simulink model "YMBOX_Control_Core"  (R2024b)
settings: Solver=FixedStepDiscrete  StartTime=0.0  StopTime=3  RelTol=1e-3
PreLoadFcn:
  | run(fullfile(fileparts(get_param(bdroot,'FileName')), 'YMBOX_Deluxe_init.m'));
InitFcn:
  | YMBOX_InitializeModel('core',bdroot);
model workspace (MAT data in the model file):
  KuMDAS_ObserverBuildVariant : Simulink.Parameter (value not decoded)
undefined symbols (not defined in the file or in its folder): CeMDSM_DrvModeIfStart_enum, CeMDSM_DrvModeSpdSens_enum, CeMDSM_DrvModeSpdSmo_enum, CeMDSM_DrvModeTrq_enum, Cf_CONTROL_TASK_TIME_S, KbMDAS_SmoDeadTimeCompEnable_flg, KbMDSA_ActiveInverterCompEnable_flg, KbMDSA_UnifiedVoltageLimitEnable_flg, KbMDSP_DCBusVoltReportFilterEnable_flg, KbMDTM_DAxisPriorityInFW_flg, KbMDTM_FieldWeakeningEnable_flg, KbMDTM_FinalIqAntiWindupEnable_flg, KbMDTM_SensorlessFieldWeakeningEnable_flg, KbMDTM_TorquePriorityBelowBase_flg, KbMDTM_UnifiedConstraintEnable_flg, KfMDAS_ControlCountToElecRad_NULL, KfMDAS_IfAccel_rpms, KfMDAS_IfAlignTime_s, KfMDAS_IfBlendTime_s, KfMDAS_IfSwitchSpd_rpm, KfMDAS_NativeCountToMechRad_NULL, KfMDAS_ObserverExitRatio_NULL, KfMDAS_SlsCtrlPeriod_s, KfMDAS_SlsEAngleInit_rad, KfMDAS_SlsElecSpdMax_rads, KfMDAS_SlsElecSpdMin_rads, KfMDAS_SlsTwoPi_rad, KfMDAS_SmoAngleOffset_rad, KfMDAS_SmoCurrentZohCoefA_NULL, KfMDAS_SmoCurrentZohCoefB_AperV, KfMDAS_SmoDeadTimeCurrentBoundary_A, KfMDAS_SmoDeadTimeDuty_NULL, KfMDAS_SmoDeadTimePolarity_NULL, KfMDAS_SmoDeviceDrop_V, KfMDAS_SmoEmfLpfCoefA_NULL, KfMDAS_SmoEmfLpfCoefB_NULL, KfMDAS_SmoEmfLpfInvPole_s, KfMDAS_SmoErrBoundaryMax_A, KfMDAS_SmoErrBoundarySpan_A, KfMDAS_SmoGainSchedAlpha_NULL, KfMDAS_SmoGainSchedAngleComp_rad, KfMDAS_SmoGainSchedEmfLow_V, KfMDAS_SmoGainSchedInvSpan_PerV, KfMDAS_SmoLdMinusLq_H, KfMDAS_SmoPllKiTs_NULL, KfMDAS_SmoPllKp_NULL, KfMDAS_SmoPllMinEmf_V, KfMDAS_SmoPllSpeedLpfAlpha_NULL, KfMDAS_SmoSlideGainMin_V, KfMDAS_SmoSlideGainSpan_V, KfMDAS_SmoSwitchSpd_rpm, KfMDAS_SmoTotalDelay_s, KfMDCC_DqSoftwareOverCurrentThreshold_A, KfMDCC_PiKcTsId_NULL, KfMDCC_PiKcTsIq_NULL, KfMDCC_PiKiTsId_NULL, KfMDCC_PiKiTsIq_NULL, KfMDCC_PiKpValueId_NULL, KfMDCC_PiKpValueIq_NULL, KfMDCC_PwmFreq_Hz ... (+84)
libraries: YMBOX_SharedMath_Lib x11, spsabctoAlphaBetaZeroLib x1
(part 7 of 8)

== system YMBOX_Control_Core/MDSA/MDSA_Subsystem/PwmOutput/PwmEnable/SVM/SectorCalc/If Action Subsystem1 ==
  In2 : Inport
  In1 : Inport  Port=2
  Action Port : ActionPort  ActionPortLabel=else
  Constant : Constant  OutDataTypeStr=uint8
  Constant1 : Constant  Value=3  OutDataTypeStr=uint8
  Constant2 : Constant  Value=2  OutDataTypeStr=uint8
  Relational Operator : RelationalOperator  Operator=>  OutDataTypeStr=boolean  InputSameDT=off
  Relational Operator1 : RelationalOperator  Operator=<=  OutDataTypeStr=boolean  InputSameDT=off
  Switch : Switch  Criteria=u2 ~= 0  SaturateOnIntegerOverflow=off  InputSameDT=off
  Switch1 : Switch  Criteria=u2 ~= 0  SaturateOnIntegerOverflow=off  InputSameDT=off
  Unary Minus : UnaryMinus
  Out1 : Outport
  wires:
  Relational Operator1/1 -> Switch1/2
  Constant2/1 -> Switch1/3
  In2/1 -> Relational Operator/2, Unary Minus/1
  Switch/1 -> Out1/1
  Switch1/1 -> Switch/3
  Constant1/1 -> Switch1/1
  Unary Minus/1 -> Relational Operator1/2
  Relational Operator/1 -> Switch/2
  Constant/1 -> Switch/1
  In1/1 -> Relational Operator/1, Relational Operator1/1

== system YMBOX_Control_Core/MDSA/MDSA_Subsystem/PwmOutput/PwmEnable/SVM/T1T2CoefCalc/If Action Subsystem ==
  In1 : Inport
  In2 : Inport  Port=2
  Action Port : ActionPort  ActionPortLabel=if(u1 <= u2)
  Constant : Constant  OutDataTypeStr=single
  Out1 : Outport
  Out2 : Outport  Port=2
  Out3 : Outport  Port=3
  wires:
  Constant/1 -> Out3/1
  In2/1 -> Out2/1
  In1/1 -> Out1/1

== system YMBOX_Control_Core/MDSA/MDSA_Subsystem/PwmOutput/PwmEnable/SVM/T1T2CoefCalc/If Action Subsystem1 ==
  In1 : Inport
  In2 : Inport  Port=2
  Action Port : ActionPort  ActionPortLabel=else
  Add : Sum
  Constant : Constant  Value=KfMDSA_MaxDuty_NULL-KfMDSA_MinDuty_NULL  OutDataTypeStr=single
  Divide : Product  Inputs=**
  Divide1 : Product  Inputs=**
  Divide2 : Product  Inputs=*/
  Signal Conversion : SignalConversion  OverrideOpt=off
  Out1 : Outport
  Out2 : Outport  Port=2
  Out3 : Outport  Port=3
  wires:
  Signal Conversion/1 -> Out3/1
  Constant/1 -> Divide2/1
  Divide2/1 -> Divide/2, Divide1/2, Signal Conversion/1
  Add/1 -> Divide2/2
  Divide1/1 -> Out2/1
  Divide/1 -> Out1/1
  In2/1 -> Divide1/1, Add/2
  In1/1 -> Divide/1, Add/1

== system YMBOX_Control_Core/MDSA/MDSA_Subsystem/PwmOutput/PwmEnable/SVM/T1T2CoefCalc/Switch Case Action Subsystem ==
  VfMDSA_VoltAlpha_V : Inport
  VfMDSA_VoltBeta_V : Inport  Port=2
  VfMDSA_DCBusVolt_V : Inport  Port=3
  Action Port : ActionPort  ActionPortLabel=case [ 1 ]:
  Divide : Product  Inputs=*/
  Divide1 : Product  Inputs=*/
  Gain : Gain  Gain=1.5
  Gain1 : Gain  Gain=sqrt(3)/2
  Gain2 : Gain  Gain=sqrt(3)
  Subtract : Sum  Inputs=+-
  VfMDSA_tmpT1Coef_NULL : Outport
  VfMDSA_tmpT2Coef_NULL : Outport  Port=2
  wires:
  Gain2/1 -> Divide1/1
  Divide1/1 -> VfMDSA_tmpT2Coef_NULL/1
  Divide/1 -> VfMDSA_tmpT1Coef_NULL/1
  VfMDSA_DCBusVolt_V/1 -> Divide/2, Divide1/2
  Subtract/1 -> Divide/1
  Gain1/1 -> Subtract/2
  Gain/1 -> Subtract/1
  VfMDSA_VoltBeta_V/1 -> Gain1/1, Gain2/1
  VfMDSA_VoltAlpha_V/1 -> Gain/1

== system YMBOX_Control_Core/MDSA/MDSA_Subsystem/PwmOutput/PwmEnable/SVM/T1T2CoefCalc/Switch Case Action Subsystem1 ==
  VfMDSA_VoltAlpha_V : Inport
  VfMDSA_VoltBeta_V : Inport  Port=2
  VfMDSA_DCBusVolt_V : Inport  Port=3
  Action Port : ActionPort  ActionPortLabel=case [ 2 ]:
  Add : Sum
  Divide : Product  Inputs=*/
  Divide1 : Product  Inputs=*/
  Gain : Gain  Gain=sqrt(3)/2
  Gain1 : Gain  Gain=1.5
  Gain2 : Gain  Gain=1.5
  Gain3 : Gain  Gain=sqrt(3)/2
  Subtract : Sum  Inputs=+-
  VfMDSA_tmpT1Coef_NULL : Outport
  VfMDSA_tmpT2Coef_NULL : Outport  Port=2
  wires:
  Add/1 -> Divide1/1
  Gain3/1 -> Add/2
  Gain2/1 -> Add/1
  Gain1/1 -> Subtract/2
  Gain/1 -> Subtract/1
  Divide1/1 -> VfMDSA_tmpT2Coef_NULL/1
  Divide/1 -> VfMDSA_tmpT1Coef_NULL/1
  VfMDSA_DCBusVolt_V/1 -> Divide1/2, Divide/2
  Subtract/1 -> Divide/1
  VfMDSA_VoltBeta_V/1 -> Gain/1, Gain3/1
  VfMDSA_VoltAlpha_V/1 -> Gain1/1, Gain2/1

== system YMBOX_Control_Core/MDSA/MDSA_Subsystem/PwmOutput/PwmEnable/SVM/T1T2CoefCalc/Switch Case Action Subsystem2 ==
  VfMDSA_VoltAlpha_V : Inport
  VfMDSA_VoltBeta_V : Inport  Port=2
  VuMDSA_DCBusVolt_V : Inport  Port=3
  Action Port : ActionPort  ActionPortLabel=case [ 3 ]:
  Add : Sum
  Divide : Product  Inputs=*/
  Divide1 : Product  Inputs=*/
  Gain : Gain  Gain=sqrt(3)
  Gain1 : Gain  Gain=1.5
  Gain2 : Gain  Gain=sqrt(3)/2
  Unary Minus : UnaryMinus
  VfMDSA_tmpT1Coef_NULL : Outport
  VfMDSA_tmpT2Coef_NULL : Outport  Port=2
  wires:
  Unary Minus/1 -> Divide1/1
  Add/1 -> Unary Minus/1
  Gain/1 -> Divide/1
  Gain2/1 -> Add/2
  Gain1/1 -> Add/1
  Divide1/1 -> VfMDSA_tmpT2Coef_NULL/1
  Divide/1 -> VfMDSA_tmpT1Coef_NULL/1
  VuMDSA_DCBusVolt_V/1 -> Divide/2, Divide1/2
  VfMDSA_VoltBeta_V/1 -> Gain/1, Gain2/1
  VfMDSA_VoltAlpha_V/1 -> Gain1/1

== system YMBOX_Control_Core/MDSA/MDSA_Subsystem/PwmOutput/PwmEnable/SVM/T1T2CoefCalc/Switch Case Action Subsystem3 ==
  VfMDSA_VoltAlpha_V : Inport
  VfMDSA_VoltBeta_V : Inport  Port=2
  VfMDSA_DCBusVolt_V : Inport  Port=3
  Action Port : ActionPort  ActionPortLabel=case [ 4 ]:
  Divide : Product  Inputs=*/
  Divide1 : Product  Inputs=*/
  Gain : Gain  Gain=-sqrt(3)
  Gain1 : Gain  Gain=sqrt(3)/2
  Gain2 : Gain  Gain=1.5
  Subtract : Sum  Inputs=+-
  VfMDSA_tmpT1Coef_NULL : Outport
  VfMDSA_tmpT2Coef_NULL : Outport  Port=2
  wires:
  Subtract/1 -> Divide1/1
  Gain2/1 -> Subtract/2
  Gain1/1 -> Subtract/1
  Gain/1 -> Divide/1
  Divide1/1 -> VfMDSA_tmpT2Coef_NULL/1
  Divide/1 -> VfMDSA_tmpT1Coef_NULL/1
  VfMDSA_DCBusVolt_V/1 -> Divide/2, Divide1/2
  VfMDSA_VoltBeta_V/1 -> Gain/1, Gain1/1
  VfMDSA_VoltAlpha_V/1 -> Gain2/1

== system YMBOX_Control_Core/MDSA/MDSA_Subsystem/PwmOutput/PwmEnable/SVM/T1T2CoefCalc/Switch Case Action Subsystem4 ==
  VfMDSA_VoltAlpha_V : Inport
  VfMDSA_VoltBeta_V : Inport  Port=2
  VfMDSA_DCBusVolt_V : Inport  Port=3
  Action Port : ActionPort  ActionPortLabel=case [ 5 ]:
  Divide : Product  Inputs=*/
  Divide1 : Product  Inputs=*/
  Gain : Gain  Gain=1.5
  Gain1 : Gain  Gain=sqrt(3)/2
  Gain2 : Gain  Gain=sqrt(3)/2
  Gain3 : Gain  Gain=1.5
  Subtract : Sum
  Subtract1 : Sum  Inputs=+-
  Unary Minus : UnaryMinus
  VfMDSA_tmpT1Coef_NULL : Outport
  VfMDSA_tmpT2Coef_NULL : Outport  Port=2
  wires:
  Unary Minus/1 -> Divide/1
  Subtract1/1 -> Divide1/1
  Gain2/1 -> Subtract1/2
  Gain3/1 -> Subtract1/1
  Divide1/1 -> VfMDSA_tmpT2Coef_NULL/1
  Divide/1 -> VfMDSA_tmpT1Coef_NULL/1
  VfMDSA_DCBusVolt_V/1 -> Divide/2, Divide1/2
  Subtract/1 -> Unary Minus/1
  Gain1/1 -> Subtract/2
  Gain/1 -> Subtract/1
  VfMDSA_VoltBeta_V/1 -> Gain1/1, Gain2/1
  VfMDSA_VoltAlpha_V/1 -> Gain/1, Gain3/1

== system YMBOX_Control_Core/MDSA/MDSA_Subsystem/PwmOutput/PwmEnable/SVM/T1T2CoefCalc/Switch Case Action Subsystem5 ==
  VfMDSA_VoltAlpha_V : Inport
  VfMDSA_VoltBeta_V : Inport  Port=2
  VfMDSA_DCBusVolt_V : Inport  Port=3
  Action Port : ActionPort  ActionPortLabel=case [ 6 ]:
  Divide : Product  Inputs=*/
  Divide1 : Product  Inputs=*/
  Gain : Gain  Gain=1.5
  Gain1 : Gain  Gain=sqrt(3)/2
  Gain2 : Gain  Gain=-sqrt(3)
  Subtract : Sum
  VfMDSA_tmpT1Coef_NULL : Outport
  VfMDSA_tmpT2Coef_NULL : Outport  Port=2
  wires:
  Gain2/1 -> Divide1/1
  Divide1/1 -> VfMDSA_tmpT2Coef_NULL/1
  Divide/1 -> VfMDSA_tmpT1Coef_NULL/1
  VfMDSA_DCBusVolt_V/1 -> Divide/2, Divide1/2
  Subtract/1 -> Divide/1
  Gain1/1 -> Subtract/2
  Gain/1 -> Subtract/1
  VfMDSA_VoltBeta_V/1 -> Gain1/1, Gain2/1
  VfMDSA_VoltAlpha_V/1 -> Gain/1

== system YMBOX_Control_Core/MDSA/MDSA_Subsystem/PwmOutput/PwmEnable/SVM/TonUVWCal/Switch Case Action Subsystem ==
  VfMDSA_PwmDutyCyclePhaseA_NULL : Inport
  VfMDSA_PwmDutyCyclePhaseB_NULL : Inport  Port=2
  VfMDSA_PwmDutyCyclePhaseC_NULL : Inport  Port=3
  Action Port : ActionPort  ActionPortLabel=case [ 1 ]:
  VfMDSA_PwmDutyCyclePhaseU_NULL : Outport
  VfMDSA_PwmDutyCyclePhaseV_NULL : Outport  Port=2
  VfMDSA_PwmDutyCyclePhaseW_NULL : Outport  Port=3
  wires:
  VfMDSA_PwmDutyCyclePhaseC_NULL/1 -> VfMDSA_PwmDutyCyclePhaseW_NULL/1
  VfMDSA_PwmDutyCyclePhaseB_NULL/1 -> VfMDSA_PwmDutyCyclePhaseV_NULL/1
  VfMDSA_PwmDutyCyclePhaseA_NULL/1 -> VfMDSA_PwmDutyCyclePhaseU_NULL/1

== system YMBOX_Control_Core/MDSA/MDSA_Subsystem/PwmOutput/PwmEnable/SVM/TonUVWCal/Switch Case Action Subsystem1 ==
  VfMDSA_PwmDutyCyclePhaseA_NULL : Inport
  VfMDSA_PwmDutyCyclePhaseB_NULL : Inport  Port=2
  VfMDSA_PwmDutyCyclePhaseC_NULL1 : Inport  Port=3
  Action Port : ActionPort  ActionPortLabel=case [ 2 ]:
  VfMDSA_PwmDutyCyclePhaseU_NULL : Outport
  VfMDSA_PwmDutyCyclePhaseV_NULL : Outport  Port=2
  VfMDSA_PwmDutyCyclePhaseW_NULL : Outport  Port=3
  wires:
  VfMDSA_PwmDutyCyclePhaseA_NULL/1 -> VfMDSA_PwmDutyCyclePhaseV_NULL/1
  VfMDSA_PwmDutyCyclePhaseB_NULL/1 -> VfMDSA_PwmDutyCyclePhaseU_NULL/1
  VfMDSA_PwmDutyCyclePhaseC_NULL1/1 -> VfMDSA_PwmDutyCyclePhaseW_NULL/1

== system YMBOX_Control_Core/MDSA/MDSA_Subsystem/PwmOutput/PwmEnable/SVM/TonUVWCal/Switch Case Action Subsystem2 ==
  VfMDSA_PwmDutyCyclePhaseA_NULL : Inport
  VfMDSA_PwmDutyCyclePhaseB_NULL : Inport  Port=2
  VfMDSA_PwmDutyCyclePhaseC_NULL : Inport  Port=3
  Action Port : ActionPort  ActionPortLabel=case [ 3 ]:
  VfMDSA_PwmDutyCyclePhaseU_NULL : Outport
  VfMDSA_PwmDutyCyclePhaseV_NULL : Outport  Port=2
  VfMDSA_PwmDutyCyclePhaseW_NULL : Outport  Port=3
  wires:
  VfMDSA_PwmDutyCyclePhaseB_NULL/1 -> VfMDSA_PwmDutyCyclePhaseW_NULL/1
  VfMDSA_PwmDutyCyclePhaseA_NULL/1 -> VfMDSA_PwmDutyCyclePhaseV_NULL/1
  VfMDSA_PwmDutyCyclePhaseC_NULL/1 -> VfMDSA_PwmDutyCyclePhaseU_NULL/1

== system YMBOX_Control_Core/MDSA/MDSA_Subsystem/PwmOutput/PwmEnable/SVM/TonUVWCal/Switch Case Action Subsystem3 ==
  VfMDSA_PwmDutyCyclePhaseA_NULL : Inport
  VfMDSA_PwmDutyCyclePhaseB_NULL : Inport  Port=2
  VfMDSA_PwmDutyCyclePhaseC_NULL : Inport  Port=3
  Action Port : ActionPort  ActionPortLabel=case [ 4 ]:
  VfMDSA_PwmDutyCyclePhaseU_NULL : Outport
  VfMDSA_PwmDutyCyclePhaseV_NULL : Outport  Port=2
  VfMDSA_PwmDutyCyclePhaseW_NULL : Outport  Port=3
  wires:
  VfMDSA_PwmDutyCyclePhaseA_NULL/1 -> VfMDSA_PwmDutyCyclePhaseW_NULL/1
  VfMDSA_PwmDutyCyclePhaseB_NULL/1 -> VfMDSA_PwmDutyCyclePhaseV_NULL/1
  VfMDSA_PwmDutyCyclePhaseC_NULL/1 -> VfMDSA_PwmDutyCyclePhaseU_NULL/1

== system YMBOX_Control_Core/MDSA/MDSA_Subsystem/PwmOutput/PwmEnable/SVM/TonUVWCal/Switch Case Action Subsystem4 ==
  VfMDSA_PwmDutyCyclePhaseA_NULL : Inport
  VfMDSA_PwmDutyCyclePhaseB_NULL : Inport  Port=2
  VfMDSA_PwmDutyCyclePhaseC_NULL : Inport  Port=3
  Action Port : ActionPort  ActionPortLabel=case [ 5 ]:
  VfMDSA_PwmDutyCyclePhaseU_NULL : Outport
  VfMDSA_PwmDutyCyclePhaseV_NULL : Outport  Port=2
  VfMDSA_PwmDutyCyclePhaseW_NULL : Outport  Port=3
  wires:
  VfMDSA_PwmDutyCyclePhaseA_NULL/1 -> VfMDSA_PwmDutyCyclePhaseW_NULL/1
  VfMDSA_PwmDutyCyclePhaseC_NULL/1 -> VfMDSA_PwmDutyCyclePhaseV_NULL/1
  VfMDSA_PwmDutyCyclePhaseB_NULL/1 -> VfMDSA_PwmDutyCyclePhaseU_NULL/1

== system YMBOX_Control_Core/MDSA/MDSA_Subsystem/PwmOutput/PwmEnable/SVM/TonUVWCal/Switch Case Action Subsystem5 ==
  VfMDSA_PwmDutyCyclePhaseA_NULL : Inport
  VfMDSA_PwmDutyCyclePhaseB_NULL : Inport  Port=2
  VfMDSA_PwmDutyCyclePhaseC_NULL : Inport  Port=3
  Action Port : ActionPort  ActionPortLabel=case [ 6 ]:
  VfMDSA_PwmDutyCyclePhaseU_NULL : Outport
  VfMDSA_PwmDutyCyclePhaseV_NULL : Outport  Port=2
  VfMDSA_PwmDutyCyclePhaseW_NULL : Outport  Port=3
  wires:
  VfMDSA_PwmDutyCyclePhaseB_NULL/1 -> VfMDSA_PwmDutyCyclePhaseW_NULL/1
  VfMDSA_PwmDutyCyclePhaseC_NULL/1 -> VfMDSA_PwmDutyCyclePhaseV_NULL/1
  VfMDSA_PwmDutyCyclePhaseA_NULL/1 -> VfMDSA_PwmDutyCyclePhaseU_NULL/1

== stateflow chart YMBOX_Control_Core/Control_Task_Dispatcher/Scheduler ==
  settings: sampleTime=50e-6
  (default) -> (junction 78) : {
      |   trig_MDSP_ControlTask;
      |   trig_MDFM_ControlTask;
      |   trig_MDSM_ControlTask;
      |   trig_MDAS_ControlTask;
      |   VuMDTM_DividerCount_NULL = VuMDTM_DividerCount_NULL + 1;
      | }
  (junction 78) -> (junction 80) [order 2]
  (junction 78) -> (junction 79) [order 1] : [VuMDTM_DividerCount_NULL >= KuMDTM_TaskDivider_NULL || MDTM_ResetDispatch]
      | {
      |  VuMDTM_DividerCount_NULL = 0;
      |  trig_MDTM_ControlTask;
      | }
  (junction 80) -> (junction 68) : {
      |   trig_MDCC_ControlTask;
      |   trig_MDSA_ControlTask;
      | }
  (junction 79) -> (junction 68) : {
      |   trig_MDCC_ControlTask;
      |   trig_MDSA_ControlTask;
      | }
  data: KuMDTM_TaskDivider_NULL parameter uint16; VuMDTM_DividerCount_NULL local uint16; MDTM_ResetDispatch data_store_memory
  events: trig_MDFM_ControlTask output FUNCTION_CALL_EVENT; trig_MDSM_ControlTask output FUNCTION_CALL_EVENT; trig_MDAS_ControlTask output FUNCTION_CALL_EVENT; trig_MDTM_ControlTask output FUNCTION_CALL_EVENT; trig_MDCC_ControlTask output FUNCTION_CALL_EVENT; trig_MDSA_ControlTask output FUNCTION_CALL_EVENT; trig_MDSP_ControlTask output FUNCTION_CALL_EVENT

== stateflow chart YMBOX_Control_Core/MDSM/MDSM_ModeManager/MDSM_Supervisor_Variant/MDSM_Supervisor_SMO/MDSM_GenericSupervisor ==
  settings: description=INDUSTRIAL_SENSORLESS_V6. Generic runtime supervisor. The compile-time Variant route table supplies observer identity, qualification, threshold, acquisition dwell and optional fallback. Stateflow only supervises I/F, STAGE1 and optional STAGE2.
  state OFF
    entry:
    VeMDSM_DrvModeCmd_enum=0; VuMDSM_StateDwell_cnt=0;
    VbMDTM_PiReset_flg=1; VbMDCC_PiReset_flg=1; VuMDFM_FFEnable_enum=0;
    during:
    VeMDSM_DrvModeCmd_enum=0; VuMDSM_StateDwell_cnt=0;
    VbMDTM_PiReset_flg=0; VbMDCC_PiReset_flg=0; VuMDFM_FFEnable_enum=0;
  state DIRECT
    entry:
    VeMDSM_ActiveDirectMode_enum=VeMDSM_DrvModeReq_enum;
    VeMDSM_DrvModeCmd_enum=VeMDSM_ActiveDirectMode_enum; VuMDSM_StateDwell_cnt=0;
    VbMDTM_PiReset_flg=1; VbMDCC_PiReset_flg=1; VuMDFM_FFEnable_enum=(VeMDSM_ActiveDirectMode_enum>=3)*KuMDCC_VoltageFFMode_enum;
    during:
    VbMDTM_PiReset_flg=(VeMDSM_DrvModeReq_enum!=VeMDSM_ActiveDirectMode_enum);
    VbMDCC_PiReset_flg=VbMDTM_PiReset_flg;
    VeMDSM_ActiveDirectMode_enum=VeMDSM_DrvModeReq_enum;
    VeMDSM_DrvModeCmd_enum=VeMDSM_ActiveDirectMode_enum; VuMDSM_StateDwell_cnt=0; VuMDFM_FFEnable_enum=(VeMDSM_ActiveDirectMode_enum>=3)*KuMDCC_VoltageFFMode_enum;
  state SENSORLESS
    state IF_RAMP
      entry:
      VeMDSM_DrvModeCmd_enum=16; VuMDSM_StateDwell_cnt=0; VuMDFM_FFEnable_enum=KuMDCC_VoltageFFMode_enum;
      during:
      VeMDSM_DrvModeCmd_enum=16;
      VuMDSM_StateDwell_cnt=VuMDSM_StateDwell_cnt+1;
      VbMDTM_PiReset_flg=0; VbMDCC_PiReset_flg=0; VuMDFM_FFEnable_enum=KuMDCC_VoltageFFMode_enum;
    state SMO_ACTIVE
      entry:
      VeMDSM_DrvModeCmd_enum=VeMDSM_Stage1Mode_enum; VuMDSM_StateDwell_cnt=0;
      VuMDSM_AcquireElapsed_cnt=VuMDSM_AcquireElapsed_cnt+(VuMDSM_AcquireElapsed_cnt<VuMDSM_Stage1Acquire_cnt);
      VuMDFM_FFEnable_enum=KuMDCC_VoltageFFMode_enum;
      during:
      VeMDSM_DrvModeCmd_enum=VeMDSM_Stage1Mode_enum;
      VuMDSM_AcquireElapsed_cnt=VuMDSM_AcquireElapsed_cnt+(VuMDSM_AcquireElapsed_cnt<VuMDSM_Stage1Acquire_cnt);
      VbMDTM_PiReset_flg=0; VbMDCC_PiReset_flg=0; VuMDFM_FFEnable_enum=KuMDCC_VoltageFFMode_enum;
    state SMO_LOSS_CONFIRM
      entry:
      VeMDSM_DrvModeCmd_enum=VeMDSM_Stage1Mode_enum; VuMDSM_StateDwell_cnt=1;
      VuMDSM_AcquireElapsed_cnt=VuMDSM_AcquireElapsed_cnt+(VuMDSM_AcquireElapsed_cnt<VuMDSM_Stage1Acquire_cnt);
      VbMDTM_PiReset_flg=0; VbMDCC_PiReset_flg=0; VuMDFM_FFEnable_enum=KuMDCC_VoltageFFMode_enum;
      during:
      VeMDSM_DrvModeCmd_enum=VeMDSM_Stage1Mode_enum;
      VuMDSM_StateDwell_cnt=VuMDSM_StateDwell_cnt+(VuMDSM_StateDwell_cnt<KuMDSM_ObserverLossConfirmCnt);
      VuMDSM_AcquireElapsed_cnt=VuMDSM_AcquireElapsed_cnt+(VuMDSM_AcquireElapsed_cnt<VuMDSM_Stage1Acquire_cnt);
      VbMDTM_PiReset_flg=0; VbMDCC_PiReset_flg=0; VuMDFM_FFEnable_enum=KuMDCC_VoltageFFMode_enum;
    state SENSORLESS_FAULT
      entry:
      VeMDSM_DrvModeCmd_enum=0; VuMDSM_StateDwell_cnt=0;
      VbMDTM_PiReset_flg=1; VbMDCC_PiReset_flg=1; VuMDFM_FFEnable_enum=0;
      during:
      VeMDSM_DrvModeCmd_enum=0; VuMDSM_StateDwell_cnt=0;
      VbMDTM_PiReset_flg=0; VbMDCC_PiReset_flg=0; VuMDFM_FFEnable_enum=0;
    state IF_LOW_SPEED
      entry:
      VeMDSM_DrvModeCmd_enum=16; VuMDSM_StateDwell_cnt=0;
      VbMDTM_PiReset_flg=1; VbMDCC_PiReset_flg=1; VuMDFM_FFEnable_enum=KuMDCC_VoltageFFMode_enum;
      during:
      VeMDSM_DrvModeCmd_enum=16; VuMDSM_StateDwell_cnt=0;
      VbMDTM_PiReset_flg=0; VbMDCC_PiReset_flg=0; VuMDFM_FFEnable_enum=KuMDCC_VoltageFFMode_enum;
    (default) -> IF_RAMP : /VbMDTM_PiReset_flg=1; VbMDCC_PiReset_flg=1;
    IF_RAMP -> SENSORLESS_FAULT [order 3] : [abs(VfMDSM_TrgtSpd_rpm)>=VfMDSM_Stage1SwitchSpd_rpm && VbMDSM_Stage1Ready_flg==0 && VuMDSM_StateDwell_cnt>=KuMDSM_IFStartupTimeoutCnt]
    IF_RAMP -> SMO_ACTIVE [order 2] : [abs(VfMDSM_TrgtSpd_rpm)>=VfMDSM_Stage1SwitchSpd_rpm && VbMDSM_Stage1Ready_flg!=0]/VuMDSM_AcquireElapsed_cnt=0; VbMDTM_PiReset_flg=1; VbMDCC_PiReset_flg=0;
    SMO_LOSS_CONFIRM -> IF_RAMP [order 3] : [VuMDSM_StateDwell_cnt>=KuMDSM_ObserverLossConfirmCnt && VuMDSM_AcquireElapsed_cnt<VuMDSM_Stage1Acquire_cnt]/VbMDTM_PiReset_flg=0; VbMDCC_PiReset_flg=0;
    IF_RAMP -> IF_LOW_SPEED [order 1] : [abs(VfMDSM_TrgtSpd_rpm)<VfMDSM_Stage1SwitchSpd_rpm]
    IF_LOW_SPEED -> IF_RAMP : [abs(VfMDSM_TrgtSpd_rpm)>=VfMDSM_Stage1SwitchSpd_rpm]/VbMDTM_PiReset_flg=0; VbMDCC_PiReset_flg=0;
    SMO_ACTIVE -> SMO_LOSS_CONFIRM : [VbMDSM_Stage1Ready_flg==0]
    SMO_LOSS_CONFIRM -> SMO_ACTIVE [order 1] : [VbMDSM_Stage1Ready_flg!=0]/VbMDTM_PiReset_flg=0; VbMDCC_PiReset_flg=0;
    SMO_LOSS_CONFIRM -> SENSORLESS_FAULT [order 4] : [VuMDSM_StateDwell_cnt>=KuMDSM_ObserverLossConfirmCnt && VuMDSM_AcquireElapsed_cnt>=VuMDSM_Stage1Acquire_cnt]
    SMO_LOSS_CONFIRM -> IF_LOW_SPEED [order 2] : [VuMDSM_StateDwell_cnt>=KuMDSM_ObserverLossConfirmCnt && abs(VfMDSM_TrgtSpd_rpm)<KfMDAS_ObserverExitRatio_NULL*VfMDSM_Stage1SwitchSpd_rpm]
  (default) -> OFF
  DIRECT -> OFF [order 1] : [VbMDSM_MCUEnb_flg==0 || VeMDSM_DrvModeReq_enum==0 || VeMDSM_DrvModeReq_enum>6]
  OFF -> DIRECT [order 1] : [VbMDSM_MCUEnb_flg!=0 && VeMDSM_DrvModeReq_enum>=1 && VeMDSM_DrvModeReq_enum<=5]
  SENSORLESS -> OFF [order 1] : [VbMDSM_MCUEnb_flg==0 || VeMDSM_DrvModeReq_enum==0 || VeMDSM_DrvModeReq_enum>6]
  OFF -> SENSORLESS [order 2] : [VbMDSM_MCUEnb_flg!=0 && VeMDSM_DrvModeReq_enum==6]
  SENSORLESS -> DIRECT [order 2] : [VbMDSM_MCUEnb_flg!=0 && VeMDSM_DrvModeReq_enum>=1 && VeMDSM_DrvModeReq_enum<=5]
  DIRECT -> SENSORLESS [order 2] : [VbMDSM_MCUEnb_flg!=0 && VeMDSM_DrvModeReq_enum==6]
  data: VeMDSM_DrvModeReq_enum input; VbMDSM_MCUEnb_flg input; VbMDSM_RouteSupported_flg input; VeMDSM_Stage1Mode_enum input; VbMDSM_Stage1Ready_flg input; VfMDSM_Stage1SwitchSpd_rpm input; VuMDSM_Stage1Acquire_cnt input; VbMDSM_Stage2Enable_flg input; VeMDSM_Stage2Mode_enum input; VbMDSM_Stage2Ready_flg input; VfMDSM_Stage2SwitchSpd_rpm input; VbMDSM_Stage2Fallback_flg input; VfMDSM_TrgtSpd_rpm input; VeMDSM_DrvModeCmd_enum output uint16; VbMDTM_PiReset_flg output boolean; VbMDCC_PiReset_flg output boolean; VuMDFM_FFEnable_enum output uint8; KuMDSM_ObserverLossConfirmCnt parameter uint32; KuMDSM_IFStartupTimeoutCnt parameter uint32; KfMDAS_ObserverExitRatio_NULL parameter single; VeMDSM_ActiveDirectMode_enum local uint16; VuMDSM_StateDwell_cnt local uint32; KuMDCC_VoltageFFMode_enum parameter uint8; VuMDSM_AcquireElapsed_cnt local uint32

== stateflow chart YMBOX_Control_Core/MDAS/IF_Startup_Internal/IF_Startup_SMO/SMO_ProductMode_Core ==
  state RunSMOProductMode
    en:
    [VfMDAS_IfMechSpd_rads, VfMDAS_IfMechSpdAbs_rads, ...
    VfMDAS_IfElecAngle_rad, VfMDAS_SmoMechSpd_rads, ...
    VfMDAS_SmoMechSpdAbs_rads, VbMDAS_SmoReady_flg, ...
    VfMDAS_SmoAlignedElecAngle_rad, VfMDAS_HandoverBlend_NULL, ...
    VfMDAS_HandoverElecAngleDelta_rad] = YMBOX_SmoProductModeCore( ...
    VeMDAS_DrvModeCmd_enum, VeMDAS_DrvModeReq_enum, ...
    VfMDAS_TargetSpd_rpm, VfMDAS_SmoElecSpd_rads, ...
    VfMDAS_SmoElecAngle_rad, VfMDAS_SmoEmfMag_V, ...
    VfMDAS_SmoPllPhaseErr_NULL, KfMDAS_SlsCtrlPeriod_s, ...
    KuMDMP_Pole_Pair_Number_NULL, KfMDAS_IfAccel_rpms, ...
    KfMDAS_IfAccelBlendTime_s, KfMDAS_IfAlignTime_s, ...
    KfMDAS_IfBlendTime_s, KfMDAS_SmoSwitchSpd_rpm, ...
    KfMDAS_SmoReadySpdErr_rads, KfMDAS_SmoReadyPllErr_NULL, ...
    KuMDAS_SmoReadyConfirmCnt, KfMDAS_SmoPllMinEmf_V, ...
    KfMDAS_DirectHandoverTime_s, KfMDAS_ObserverExitRatio_NULL);
    du:
    [VfMDAS_IfMechSpd_rads, VfMDAS_IfMechSpdAbs_rads, ...
    VfMDAS_IfElecAngle_rad, VfMDAS_SmoMechSpd_rads, ...
    VfMDAS_SmoMechSpdAbs_rads, VbMDAS_SmoReady_flg, ...
    VfMDAS_SmoAlignedElecAngle_rad, VfMDAS_HandoverBlend_NULL, ...
    VfMDAS_HandoverElecAngleDelta_rad] = YMBOX_SmoProductModeCore( ...
    VeMDAS_DrvModeCmd_enum, VeMDAS_DrvModeReq_enum, ...
    VfMDAS_TargetSpd_rpm, VfMDAS_SmoElecSpd_rads, ...
    VfMDAS_SmoElecAngle_rad, VfMDAS_SmoEmfMag_V, ...
    VfMDAS_SmoPllPhaseErr_NULL, KfMDAS_SlsCtrlPeriod_s, ...
    KuMDMP_Pole_Pair_Number_NULL, KfMDAS_IfAccel_rpms, ...
    KfMDAS_IfAccelBlendTime_s, KfMDAS_IfAlignTime_s, ...
    KfMDAS_IfBlendTime_s, KfMDAS_SmoSwitchSpd_rpm, ...
    KfMDAS_SmoReadySpdErr_rads, KfMDAS_SmoReadyPllErr_NULL, ...
    KuMDAS_SmoReadyConfirmCnt, KfMDAS_SmoPllMinEmf_V, ...
    KfMDAS_DirectHandoverTime_s, KfMDAS_ObserverExitRatio_NULL);
  (default) -> RunSMOProductMode
  data: VeMDAS_DrvModeCmd_enum input uint16; VeMDAS_DrvModeReq_enum input uint16; VfMDAS_TargetSpd_rpm input single; VfMDAS_SmoElecSpd_rads input single; VfMDAS_SmoElecAngle_rad input single; VfMDAS_SmoEmfMag_V input single; VfMDAS_SmoPllPhaseErr_NULL input single; VfMDAS_IfMechSpd_rads output single; VfMDAS_IfMechSpdAbs_rads output single; VfMDAS_IfElecAngle_rad output single; VfMDAS_SmoMechSpd_rads output single; VfMDAS_SmoMechSpdAbs_rads output single; VbMDAS_SmoReady_flg output boolean; VfMDAS_SmoAlignedElecAngle_rad output single; VfMDAS_HandoverBlend_NULL output single; VfMDAS_HandoverElecAngleDelta_rad output single; KfMDAS_SlsCtrlPeriod_s parameter single; KuMDMP_Pole_Pair_Number_NULL parameter uint16; KfMDAS_IfAccel_rpms parameter single; KfMDAS_IfAccelBlendTime_s parameter single; KfMDAS_IfAlignTime_s parameter single; KfMDAS_IfBlendTime_s parameter single; KfMDAS_SmoSwitchSpd_rpm parameter single; KfMDAS_SmoReadySpdErr_rads parameter single; KfMDAS_SmoReadyPllErr_NULL parameter single; KuMDAS_SmoReadyConfirmCnt parameter uint16; KfMDAS_SmoPllMinEmf_V parameter single; KfMDAS_DirectHandoverTime_s parameter single; KfMDAS_ObserverExitRatio_NULL parameter single

== matlab function YMBOX_Control_Core/MDSM/MDSM_ModeManager/MDSM_Supervisor_Variant/MDSM_Supervisor_SensoredOnly/SensoredOnly_Supervisor ==
  data: modeReq input; modeCmd output; mcuEnable input; mdtmReset output; mdccReset output; ffEnable output; KuMDCC_VoltageFFMode_enum parameter uint8
function [modeCmd,mdtmReset,mdccReset,ffEnable] = SensoredOnly_Supervisor(modeReq,mcuEnable, KuMDCC_VoltageFFMode_enum)
%#codegen
request=uint16(modeReq);
if (mcuEnable~=0) && (request>=uint16(1)) && (request<=uint16(5))
    modeCmd=request;
else
    modeCmd=uint16(0);
end
persistent previousMode
if isempty(previousMode)
    previousMode=uint16(0);
end
mdtmReset=(modeCmd~=previousMode);
mdccReset=mdtmReset;
ffEnable=uint8(0);
if modeCmd>=uint16(3)
    ffEnable=KuMDCC_VoltageFFMode_enum;
end
previousMode=modeCmd;
end

== stateflow chart YMBOX_Control_Core/MDAS/Position_Feedback_Status ==
  state Run
    entry, during:
    mechAngleRad = mod(single(rawMechCount)*single(nativeToMech),single(twoPiRad));
    if mechAngleRad < single(0), mechAngleRad = mechAngleRad + twoPiRad; end
    elecAngleRad = mod(single(selectedElecAngleRad),single(twoPiRad));
    if elecAngleRad < single(0), elecAngleRad = elecAngleRad + twoPiRad; end
    angleValid = false; speedValid = false; quality = single(0);
    if modeCmd == uint16(17)
    angleValid = smoReady; speedValid = smoReady;
    if smoReady, quality = single(0.85); else, quality = single(0.20); end
    elseif modeCmd == uint16(16)
    angleValid = true; speedValid = true; quality = single(0.50);
    elseif modeCmd >= uint16(1) && modeCmd <= uint16(5)
    angleValid = true; speedValid = true; quality = single(1);
    end
    if speedValid && selectedMechSpdRads > single(1e-4), direction = int8(1); elseif speedValid && selectedMechSpdRads < single(-1e-4), direction = int8(-1); else, direction = int8(0); end
  (default) -> Run
  data: modeCmd input uint16; rawMechCount input uint32; selectedElecAngleRad input single; selectedMechSpdRads input single; smoReady input boolean; nativeToMech input single; twoPiRad input single; mechAngleRad output single; elecAngleRad output single; angleValid output boolean; speedValid output boolean; quality output single; direction output int8

== matlab function YMBOX_Control_Core/MDTM/Command_Constraint_FieldWeakening_Manager/Operating_Point_Estimator/Estimate_Operating_Point ==
  data: iqRaw input single size=1; rpmAbs output single size=1; idRaw input single size=1; speedRads input single size=1; vdc input single size=1; vdqMaxPerVdc input single size=1; rs input single size=1; ld input single size=1; lq input single size=1; pmFlux input single size=1; polePairs input uint16 size=1; omegaElec output single size=1; vmax output single size=1; utilRaw output single size=1; modeCmd input; fwAllowed input
function [rpmAbs,omegaElec,vmax,utilRaw] = Estimate_Operating_Point(iqRaw,idRaw,speedRads,vdc,vdqMaxPerVdc,rs,ld,lq,pmFlux,polePairs,modeCmd,fwAllowed)
%#codegen
rpmAbs=single(0);
omegaElec=single(0);
vmax=single(0);
utilRaw=single(0);
if uint16(modeCmd)==uint16(0)
    return;
end
rpmAbs=abs(speedRads)*single(60/(2*pi));
omegaElec=abs(speedRads)*single(polePairs);
vmax=max(single(0),vdc*vdqMaxPerVdc);
if fwAllowed && vmax>single(1e-6)
    vdEst=rs*idRaw-omegaElec*lq*iqRaw;
    vqEst=rs*iqRaw+omegaElec*(ld*idRaw+pmFlux);
    utilRaw=hypot(vdEst,vqEst)/vmax;
end
end

== matlab function YMBOX_Control_Core/MDTM/MDTM/MDTM_SMO/SMO_Handover_SeedEstimator/Handover_Seed_State_Manager ==
  data: modeCmd input; iqObserverSeed output; modeReq input; phaseU input; phaseV input; phaseW input; elecAngleDeltaRad input; iAlpha input; iBeta input; idCtrl input; iqCtrl input; iqObs input; targetSpdRpm input; ifIq input; minDriveIq input; iqLimit input; lpfAlpha input; sourceId output; sourceIq output
function [iqObserverSeed,sourceId,sourceIq] = Handover_Seed_State_Manager(modeCmd,modeReq,phaseU,phaseV,phaseW,elecAngleDeltaRad,iAlpha,iBeta,idCtrl,iqCtrl,iqObs,targetSpdRpm,ifIq,minDriveIq,iqLimit,lpfAlpha)
%#codegen
% Latch measured current during IF tracking. Squared current limits are
% the validity contract and reject non-finite values by IEEE rules.
persistent obsIqFilt sourceIdFilt sourceIqFilt storedValid prevMode prevReq;
if isempty(obsIqFilt)
    obsIqFilt=single(0);
    sourceIdFilt=single(0);
    sourceIqFilt=single(0);
    storedValid=false;
    prevMode=uint16(0);
    prevReq=uint16(0);
end
mode=uint16(modeCmd);
req=uint16(modeReq);
trackingIf=(mode==uint16(16)) && (req==uint16(6));
handoverSmo=(mode==uint16(17)) && (req==uint16(6));
if ~(trackingIf || handoverSmo)
    obsIqFilt=single(0);
    sourceIdFilt=single(0);
    sourceIqFilt=single(0);
    storedValid=false;
    iqObserverSeed=single(0);
    sourceId=single(0);
    sourceIq=single(0);
    prevMode=mode;
    prevReq=req;
    return;
end
if req~=prevReq
    obsIqFilt=single(0);
    sourceIdFilt=single(0);
    sourceIqFilt=single(0);
    storedValid=false;
end
limit=max(single(1),abs(single(iqLimit)));
if trackingIf
    iAlphaValue=single(iAlpha);
    iBetaValue=single(iBeta);
    idCtrlValue=single(idCtrl);
    iqCtrlValue=single(iqCtrl);
    iqObsValue=single(iqObs);
    vectorMagnitudeSq=iAlphaValue*iAlphaValue+iBetaValue*iBetaValue;
    controlMagnitudeSq=idCtrlValue*idCtrlValue+iqCtrlValue*iqCtrlValue;
    observerMagnitudeSq=iqObsValue*iqObsValue;
    validMagnitudeLimit=single(1.25)*limit;
    validMagnitudeLimitSq=validMagnitudeLimit*validMagnitudeLimit;
    sampleValid=(vectorMagnitudeSq<=validMagnitudeLimitSq) && ...
        (controlMagnitudeSq<=validMagnitudeLimitSq) && ...
        (observerMagnitudeSq<=validMagnitudeLimitSq);
    if sampleValid
        a=single(lpfAlpha);
        if ~storedValid || prevMode~=uint16(16)
            obsIqFilt=iqObsValue;
            sourceIdFilt=idCtrlValue;
            sourceIqFilt=iqCtrlValue;
        else
            obsIqFilt=obsIqFilt+a*(iqObsValue-obsIqFilt);
            sourceIdFilt=sourceIdFilt+a*(idCtrlValue-sourceIdFilt);
            sourceIqFilt=sourceIqFilt+a*(iqCtrlValue-sourceIqFilt);
        end
        storedValid=true;
    else
        obsIqFilt=single(0);
        sourceIdFilt=single(0);
        sourceIqFilt=single(0);
        storedValid=false;
    end
end
if storedValid
    iqTarget=obsIqFilt;
    sourceIdValue=sourceIdFilt;
    sourceIqValue=sourceIqFilt;
elseif handoverSmo
    ifIqValue=single(ifIq);
    cosDelta=MDTM_Cos_Rad_f32(single(elecAngleDeltaRad));
    fallbackIq=ifIqValue*cosDelta;
    limitSq=limit*limit;
    if ifIqValue*ifIqValue<=limitSq && fallbackIq*fallbackIq<=limitSq
        iqTarget=fallbackIq;
        sourceIdValue=single(0);
        sourceIqValue=ifIqValue;
    else
        iqTarget=single(0);
        sourceIdValue=single(0);
        sourceIqValue=single(0);
    end
else
    iqTarget=single(0);
    sourceIdValue=single(0);
    sourceIqValue=single(0);
end
direction=single(0);
if single(targetSpdRpm)>single(1e-3)
    direction=single(1);
elseif single(targetSpdRpm)<single(-1e-3)
    direction=single(-1);
end
minimum=abs(single(minDriveIq));
if direction~=single(0) && direction*iqTarget<minimum
    iqTarget=direction*minimum;
end
iqTarget=min(limit,max(-limit,iqTarget));
sourceMagnitude=sqrt(sourceIdValue*sourceIdValue+sourceIqValue*sourceIqValue);
if sourceMagnitude>limit
    scale=limit/sourceMagnitude;
    sourceIdValue=sourceIdValue*scale;
    sourceIqValue=sourceIqValue*scale;
end
iqObserverSeed=single(iqTarget);
sourceId=single(sourceIdValue);
sourceIq=single(sourceIqValue);
prevMode=mode;
prevReq=req;
% phaseU/V/W remain only for compatibility with the published interface.
end

function cosTheta=MDTM_Cos_Rad_f32(thetaRad)
coder.inline('always');
anglePu=single(thetaRad)*single(0.1591549);
anglePu=anglePu-floor(anglePu);
cosTheta=single(0);
sinTheta=single(0);
coder.cinclude('mdsa_sincos_f32.h');
coder.ceval('MDSA_SinCos_f32',anglePu,coder.wref(cosTheta),coder.wref(sinTheta));
end

== matlab function YMBOX_Control_Core/MDTM/Command_Constraint_FieldWeakening_Manager/Field_Weakening_Controller/Field_Weakening_State_Update ==
  data: idRaw input single size=1; fwStateNext output boolean size=1; iqRaw input single size=1; rpmAbs input single size=1; omegaElec input single size=1; vmax input single size=1; utilRaw input single size=1; fwAllowed input boolean size=1; modeCmd input uint16 size=1; ld input single size=1; lq input single size=1; pmFlux input single size=1; fwEntryUtil input single size=1; fwExitUtil input single size=1; fwEntrySpeedRpm input single size=1; fwIdMin input single size=1; fwKp input single size=1; fwKiTs input single size=1; fwIdSlew input single size=1; fwStatePrev input boolean size=1; fwIntegratorPrev input single size=1; fwIdStatePrev input single size=1; fwIntegratorNext output single size=1; fwIdStateNext output single size=1; idRequest output single size=1; fwActive output boolean size=1; fwIdContribution output single size=1
function [fwStateNext,fwIntegratorNext,fwIdStateNext,idRequest,fwActive,fwIdContribution] = Field_Weakening_State_Update(idRaw,iqRaw,rpmAbs,omegaElec,vmax,utilRaw,fwAllowed,modeCmd,ld,lq,pmFlux,fwEntryUtil,fwExitUtil,fwEntrySpeedRpm,fwIdMin,fwKp,fwKiTs,fwIdSlew,fwStatePrev,fwIntegratorPrev,fwIdStatePrev)
%#codegen
if uint16(modeCmd)==uint16(0)
    fwStateNext=false;
    fwIntegratorNext=single(0);
    fwIdStateNext=single(0);
    idRequest=single(0);
    fwActive=false;
    fwIdContribution=single(0);
    return;
end
fwStateNext=logical(fwStatePrev);
fwIntegratorNext=single(fwIntegratorPrev);
fwIdStateNext=single(fwIdStatePrev);
idTarget=single(0);
if ~fwAllowed
    fwStateNext=false; fwIntegratorNext=single(0); fwIdStateNext=single(0);
else
    if ~fwStateNext && ((rpmAbs>=single(0.8)*fwEntrySpeedRpm && utilRaw>=fwEntryUtil) || rpmAbs>=fwEntrySpeedRpm)
        fwStateNext=true;
    end
    if fwStateNext && utilRaw<=fwExitUtil && rpmAbs<single(0.98)*fwEntrySpeedRpm
        fwStateNext=false;
    end
    if fwStateNext
        if omegaElec>single(1) && ld>single(1e-9)
            vdMagnitude=abs(omegaElec*lq*iqRaw);
            vqAvailable=sqrt(max(single(0),(vmax-vdMagnitude)*(vmax+vdMagnitude)));
            idFeedforward=single((vqAvailable/omegaElec-pmFlux)/ld);
        else
            idFeedforward=single(0);
        end
        idFeedforward=single(min(single(0),max(fwIdMin,idFeedforward)));
        fwError=single(utilRaw-fwEntryUtil);
        fwIntegratorNext=single(min(single(0),max(fwIdMin,fwIntegratorPrev-fwKiTs*fwError)));
        idPi=single(min(single(0),max(fwIdMin,fwIntegratorNext-fwKp*max(single(0),fwError))));
        idTarget=min(idFeedforward,idPi);
    else
        fwIntegratorNext=single(0);
    end
    deltaId=single(min(fwIdSlew,max(-fwIdSlew,idTarget-fwIdStatePrev)));
    fwIdStateNext=single(fwIdStatePrev+deltaId);
end
fwActive=fwStateNext || fwIdStateNext<single(-1e-4);
fwIdContribution=fwIdStateNext;
idRequest=single(idRaw);
if fwActive
    idRequest=single(min(idRaw,fwIdStateNext));
end
end

== matlab function YMBOX_Control_Core/MDTM/Command_Constraint_FieldWeakening_Manager/Current_Vector_Constraint/Apply_Current_Vector_Constraint ==
  data: iqRaw input single size=1; iqCmd output single size=1; idRaw input single size=1; idRequest input single size=1; fwActive input boolean size=1; unifiedEnable input boolean size=1; currentMax input single size=1; torquePriority input boolean size=1; dAxisPriority input boolean size=1; idCmd output single size=1; iqLimit output single size=1; currentLimited output boolean size=1; modeCmd input
function [iqCmd,idCmd,iqLimit,currentLimited] = Apply_Current_Vector_Constraint(iqRaw,idRaw,idRequest,fwActive,unifiedEnable,currentMax,torquePriority,dAxisPriority,modeCmd)
%#codegen
iqCmd=single(0);
idCmd=single(0);
iqLimit=single(0);
currentLimited=false;
if uint16(modeCmd)==uint16(0)
    return;
end
iqCmd=single(iqRaw);
idCmd=single(idRequest);
iqLimit=max(single(0),single(currentMax));
if unifiedEnable && currentMax>single(0)
    if fwActive && dAxisPriority
        idCmd=single(min(currentMax,max(-currentMax,idRequest)));
        iqLimit=single(remainingAxisLimit(currentMax,idCmd));
        iqCmd=single(min(iqLimit,max(-iqLimit,iqRaw)));
    elseif torquePriority
        iqCmd=single(min(currentMax,max(-currentMax,iqRaw)));
        idLimit=single(remainingAxisLimit(currentMax,iqCmd));
        idCmd=single(min(idLimit,max(-idLimit,idRequest)));
        iqLimit=single(currentMax);
    else
        idCmd=single(min(currentMax,max(-currentMax,idRequest)));
        iqLimit=single(remainingAxisLimit(currentMax,idCmd));
        iqCmd=single(min(iqLimit,max(-iqLimit,iqRaw)));
    end
    currentLimited=abs(iqCmd-iqRaw)>single(1e-5) || abs(idCmd-idRaw)>single(1e-5);
end
end

function axisLimit=remainingAxisLimit(currentMax,axisCmd)
% Factor the difference of squares to retain accuracy near the current limit.
axisAbs=abs(axisCmd);
axisLimit=sqrt(max(single(0),(currentMax-axisAbs)*(currentMax+axisAbs)));
end

== matlab function YMBOX_Control_Core/MDTM/MDTM/MDTM_SMO/Action_IF_Startup/IF_Current_Profile ==
  data: speedCmdRpm input; iqCmd output; resetFlag input; Ts input; alignTime input; blendTime input; alignId input; runIq input; iqSlew input; idCmd output
function [iqCmd,idCmd] = IF_Current_Profile(speedCmdRpm,resetFlag,Ts,alignTime,blendTime,alignId,runIq,iqSlew)
%#codegen
coder.cinclude('mdsa_sincos_f32.h');
persistent elapsed iqState;
if isempty(elapsed)
    elapsed=0.0; iqState=single(0);
end
% Preserve timer precision and transition samples; math outputs use single.
ts=max(1e-7,double(Ts));
if resetFlag~=0
    elapsed=0.0; iqState=single(0);
end
if speedCmdRpm==single(0)
    elapsed=0.0; iqState=single(0);
    iqCmd=single(0);
    idCmd=single(0);
    return;
end
direction=sign(speedCmdRpm);
if elapsed < max(0.0,double(alignTime))
    elapsed=elapsed+ts;
    iqState=single(0);
    iqCmd=single(0);
    idCmd=abs(alignId);
elseif elapsed < max(0.0,double(alignTime))+max(0.0,double(blendTime))
    blend=max(single(1e-7),blendTime);
    s=min(single(1),max(single(0),(single(elapsed)-alignTime)/blend));
    s=s*s*(single(3)-single(2)*s);
    magnitude=abs(alignId)+(abs(runIq)-abs(alignId))*s;
    % One quarter-turn is pi/2; call the shared board-selected SinCos API.
    anglePu=single(0.25)*s;
    cosGamma=single(0); sinGamma=single(0);
    coder.ceval('MDSA_SinCos_f32',anglePu,coder.wref(cosGamma),coder.wref(sinGamma));
    iqState=direction*magnitude*sinGamma;
    iqCmd=iqState;
    idCmd=magnitude*cosGamma;
    elapsed=elapsed+ts;
else
    targetIq=direction*abs(runIq);
    maxStep=abs(iqSlew)*single(ts);
    delta=targetIq-iqState;
    if delta>maxStep, delta=maxStep; elseif delta<-maxStep, delta=-maxStep; end
    iqState=iqState+delta;
    iqCmd=iqState;
    idCmd=single(0);
end
end

== matlab function YMBOX_Control_Core/MDTM/Command_Constraint_FieldWeakening_Manager/Command_Diagnostics/Calculate_Command_Diagnostics ==
  data: iqCmd input single size=1; currentUtilization output single size=1; idCmd input single size=1; currentMax input single size=1; omegaElec input single size=1; vmax input single size=1; rs input single size=1; ld input single size=1; lq input single size=1; pmFlux input single size=1; polePairs input uint16 size=1; voltageUtilization output single size=1; iqAntiWindupFeedback output single size=1; torqueEstimate_Nm output single size=1; modeCmd input
function [currentUtilization,voltageUtilization,iqAntiWindupFeedback,torqueEstimate_Nm] = Calculate_Command_Diagnostics(iqCmd,idCmd,currentMax,omegaElec,vmax,rs,ld,lq,pmFlux,polePairs,modeCmd)
%#codegen
currentUtilization=single(0);
voltageUtilization=single(0);
iqAntiWindupFeedback=single(0);
torqueEstimate_Nm=single(0);
if uint16(modeCmd)==uint16(0)
    return;
end
if currentMax>single(1e-6)
    currentUtilization=single(hypot(idCmd,iqCmd)/currentMax);
end
vdEst=single(rs*idCmd-omegaElec*lq*iqCmd);
vqEst=single(rs*iqCmd+omegaElec*(ld*idCmd+pmFlux));
if vmax>single(1e-6)
    voltageUtilization=single(hypot(vdEst,vqEst)/vmax);
end
torqueEstimate_Nm=single(single(1.5)*single(polePairs)*(pmFlux*iqCmd+(ld-lq)*idCmd*iqCmd));
torqueConstant=single(1.5)*single(polePairs)*pmFlux;
if abs(torqueConstant)>single(1e-9)
    iqAntiWindupFeedback=torqueEstimate_Nm/torqueConstant;
else
    iqAntiWindupFeedback=single(iqCmd);
end
end
